simulink model "ASM_AnimationInterface"  (R2024a)
settings: Solver=ode1  StartTime=SIM.tstart.v  StopTime=SIM.tend.v  FixedStep=SIM.StepSize.v  RelTol=1e-3
PostLoadFcn:
  | , if any(exist('dsrtsu_mdlpostloadfcn', 'file') ~= 0), dsrtsu_mdlpostloadfcn('Execute', bdroot); end,
undefined symbols (not defined in the file): a0b2, b98103fe8ad365046cd0, dsmsi, MDL, SIM
libraries: simulink x22, dsmsilib x15, dsmpblib x4, ASM_Environment_lib x1
(part 7 of 7)

== system ASM_AnimationInterface/AnimationInterface/ANIMATION_INTERFACE/Sensors/Line_Sensor_Road_Shape_ContObj_Points ==
  ModelSignals : Inport
  Bus Selector : BusSelector  OutputSignals=Pos_x_Road_Shape_ContObj_Animation_CoorSys_E,Pos_y_Road_Shape_ContObj_Animation_CoorSys_E,Pos_z_Road_Shape_ContObj_Animation_CoorSys_E
  CC : Concatenate  NumInputs=3  Mode=Multidimensional array
  Reshape1 : Reshape  OutputDimensionality=Row vector (2-D)
  Reshape2 : Reshape  OutputDimensionality=Row vector (2-D)
  Reshape3 : Reshape  OutputDimensionality=Row vector (2-D)
  AnimationSignals : Outport  VectorParamsAs1DForOutWhenUnconnected=off
  wires:
  ModelSignals/1 -> Bus Selector/1
  CC/1 -> AnimationSignals/1
  Bus Selector/1 -> Reshape1/1  "<Pos_x_Road_Shape_ContObj_Animation_CoorSys_E>"
  Bus Selector/2 -> Reshape2/1  "<Pos_y_Road_Shape_ContObj_Animation_CoorSys_E>"
  Bus Selector/3 -> Reshape3/1  "<Pos_z_Road_Shape_ContObj_Animation_CoorSys_E>"
  Reshape1/1 -> CC/1
  Reshape2/1 -> CC/2
  Reshape3/1 -> CC/3

== system ASM_AnimationInterface/AnimationInterface/ANIMATION_INTERFACE/Sensors/Line_Sensor_Road_Shape_Line_Points ==
  ModelSignals : Inport
  Bus Selector : BusSelector  OutputSignals=Pos_x_Road_Shape_Line_Animation_CoorSys_E,Pos_y_Road_Shape_Line_Animation_CoorSys_E,Pos_z_Road_Shape_Line_Animation_CoorSys_E
  CC : Concatenate  NumInputs=3  Mode=Multidimensional array
  Reshape1 : Reshape  OutputDimensionality=Row vector (2-D)
  Reshape2 : Reshape  OutputDimensionality=Row vector (2-D)
  Reshape3 : Reshape  OutputDimensionality=Row vector (2-D)
  AnimationSignals : Outport  VectorParamsAs1DForOutWhenUnconnected=off
  wires:
  Bus Selector/3 -> Reshape3/1  "<Pos_z_Road_Shape_Line_Animation_CoorSys_E>"
  Bus Selector/2 -> Reshape2/1  "<Pos_y_Road_Shape_Line_Animation_CoorSys_E>"
  Bus Selector/1 -> Reshape1/1  "<Pos_x_Road_Shape_Line_Animation_CoorSys_E>"
  CC/1 -> AnimationSignals/1
  ModelSignals/1 -> Bus Selector/1
  Reshape1/1 -> CC/1
  Reshape2/1 -> CC/2
  Reshape3/1 -> CC/3

== system ASM_AnimationInterface/AnimationInterface/ANIMATION_INTERFACE/Sensors/Object_Sensor_2D_Points ==
  Transform_In : Inport
  Sw_Sensor_Selector[] : Inport  Port=2
  ObjectSensor2D_1_Animation : Inport  Port=3
  ObjectSensor2D_2_Animation : Inport  Port=4
  ObjectSensor2D_3_Animation : Inport  Port=5
  ObjectSensor2D_4_Animation : Inport  Port=6
  ObjectSensor2D_5_Animation : Inport  Port=7
  ObjectSensor2D_6_Animation : Inport  Port=8
  ObjectSensor2D_7_Animation : Inport  Port=9
  Calc_Object_Sensor_2D_Points : Subsystem
  Multiport Switch : MultiPortSwitch  Inputs=7  SaturateOnIntegerOverflow=off  InputSameDT=off
  Object_Sensor_2D_Transformation1 : Subsystem
  Saturation : Saturate  UpperLimit=7  LowerLimit=1
  AnimationSignals : Outport  VectorParamsAs1DForOutWhenUnconnected=off
  wires:
  Saturation/1 -> Multiport Switch/1
  ObjectSensor2D_7_Animation/1 -> Multiport Switch/8
  ObjectSensor2D_6_Animation/1 -> Multiport Switch/7
  ObjectSensor2D_5_Animation/1 -> Multiport Switch/6
  ObjectSensor2D_4_Animation/1 -> Multiport Switch/5
  Transform_In/1 -> Object_Sensor_2D_Transformation1/1(Transform_In1)
  Object_Sensor_2D_Transformation1/1(Transform_Out) -> Calc_Object_Sensor_2D_Points/1(Transform_In)
  Calc_Object_Sensor_2D_Points/1(AnimationSignals) -> AnimationSignals/1
  ObjectSensor2D_3_Animation/1 -> Multiport Switch/4
  ObjectSensor2D_2_Animation/1 -> Multiport Switch/3
  ObjectSensor2D_1_Animation/1 -> Multiport Switch/2
  Sw_Sensor_Selector[]/1 -> Saturation/1
  Multiport Switch/1 -> Object_Sensor_2D_Transformation1/2(ModelSignals), Calc_Object_Sensor_2D_Points/2(ModelSignals)

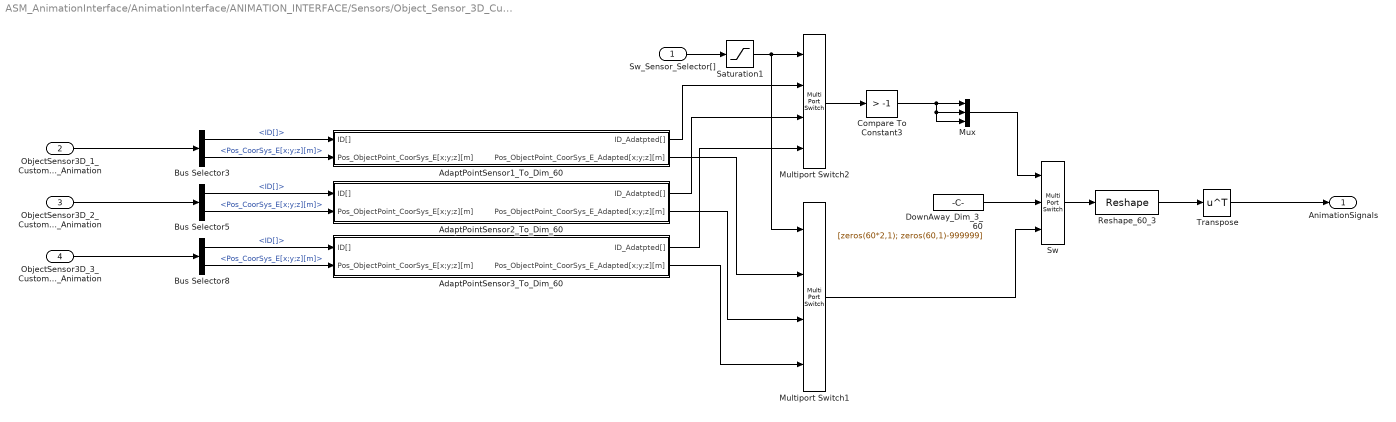
== system ASM_AnimationInterface/AnimationInterface/ANIMATION_INTERFACE/Sensors/Object_Sensor_3D_CustomPoints ==
  Sw_Sensor_Selector[] : Inport
  ObjectSensor3D_1_CustomPoints_Animation : Inport  Port=2
  ObjectSensor3D_2_CustomPoints_Animation : Inport  Port=3
  ObjectSensor3D_3_CustomPoints_Animation : Inport  Port=4
  AdaptPointSensor1_To_Dim_60 : Subsystem
  AdaptPointSensor2_To_Dim_60 : Subsystem
  AdaptPointSensor3_To_Dim_60 : Subsystem
  Bus Selector3 : BusSelector  OutputSignals=ID[],Pos_CoorSys_E[x;y;z][m]
  Bus Selector5 : BusSelector  OutputSignals=ID[],Pos_CoorSys_E[x;y;z][m]
  Bus Selector8 : BusSelector  OutputSignals=ID[],Pos_CoorSys_E[x;y;z][m]
  Compare To Constant3 : simulink/Logic and Bit Operations/Compare To Constant  relop=>  const=-1  OutDataTypeStr=boolean
  DownAway_Dim_3_60 : Constant  Value=[zeros(60*2,1); zeros(60,1)-999999]
  Multiport Switch1 : MultiPortSwitch  SaturateOnIntegerOverflow=off  InputSameDT=off
  Multiport Switch2 : MultiPortSwitch  SaturateOnIntegerOverflow=off  InputSameDT=off
  Mux : Mux  Inputs=3
  Reshape_60_3 : Reshape  OutputDimensionality=Customize  OutputDimensions=[60,3]
  Saturation1 : Saturate  UpperLimit=3  LowerLimit=1
  Sw : MultiPortSwitch  DataPortOrder=Zero-based contiguous  Inputs=2  zeroidx=on  SaturateOnIntegerOverflow=off  InputSameDT=off
  Transpose : Math  Operator=transpose  SignedPower=on
  AnimationSignals : Outport  VectorParamsAs1DForOutWhenUnconnected=off
  wires:
  Transpose/1 -> AnimationSignals/1
  AdaptPointSensor3_To_Dim_60/1(ID_Adatpted[]) -> Multiport Switch2/4
  AdaptPointSensor3_To_Dim_60/2(Pos_ObjectPoint_CoorSys_E_Adapted[x;y;z][m]) -> Multiport Switch1/4
  Multiport Switch1/1 -> Sw/3
  Bus Selector8/2 -> AdaptPointSensor3_To_Dim_60/2(Pos_ObjectPoint_CoorSys_E[x;y;z][m])  "<Pos_CoorSys_E[x;y;z][m]>"
  Bus Selector5/2 -> AdaptPointSensor2_To_Dim_60/2(Pos_ObjectPoint_CoorSys_E[x;y;z][m])  "<Pos_CoorSys_E[x;y;z][m]>"
  Bus Selector5/1 -> AdaptPointSensor2_To_Dim_60/1(ID[])  "<ID[]>"
  Multiport Switch2/1 -> Compare To Constant3/1
  Reshape_60_3/1 -> Transpose/1
  ObjectSensor3D_2_CustomPoints_Animation/1 -> Bus Selector5/1
  ObjectSensor3D_3_CustomPoints_Animation/1 -> Bus Selector8/1
  Bus Selector3/1 -> AdaptPointSensor1_To_Dim_60/1(ID[])  "<ID[]>"
  Bus Selector3/2 -> AdaptPointSensor1_To_Dim_60/2(Pos_ObjectPoint_CoorSys_E[x;y;z][m])  "<Pos_CoorSys_E[x;y;z][m]>"
  ObjectSensor3D_1_CustomPoints_Animation/1 -> Bus Selector3/1
  AdaptPointSensor1_To_Dim_60/1(ID_Adatpted[]) -> Multiport Switch2/2
  AdaptPointSensor1_To_Dim_60/2(Pos_ObjectPoint_CoorSys_E_Adapted[x;y;z][m]) -> Multiport Switch1/2
  Bus Selector8/1 -> AdaptPointSensor3_To_Dim_60/1(ID[])  "<ID[]>"
  Mux/1 -> Sw/1
  Compare To Constant3/1 -> Mux/3, Mux/2, Mux/1
  Sw_Sensor_Selector[]/1 -> Saturation1/1
  DownAway_Dim_3_60/1 -> Sw/2
  Saturation1/1 -> Multiport Switch1/1, Multiport Switch2/1
  Sw/1 -> Reshape_60_3/1
  AdaptPointSensor2_To_Dim_60/2(Pos_ObjectPoint_CoorSys_E_Adapted[x;y;z][m]) -> Multiport Switch1/3
  AdaptPointSensor2_To_Dim_60/1(ID_Adatpted[]) -> Multiport Switch2/3

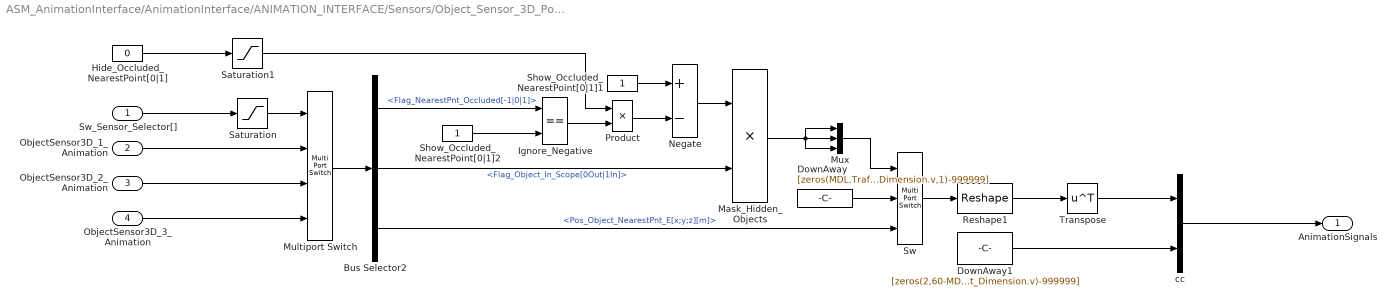
== system ASM_AnimationInterface/AnimationInterface/ANIMATION_INTERFACE/Sensors/Object_Sensor_3D_Points ==
  Sw_Sensor_Selector[] : Inport
  ObjectSensor3D_1_Animation : Inport  Port=2
  ObjectSensor3D_2_Animation : Inport  Port=3
  ObjectSensor3D_3_Animation : Inport  Port=4
  Bus Selector2 : BusSelector  OutputSignals=Flag_NearestPnt_Occluded[-1|0|1],Flag_Object_In_Scope[0Out|1In],Pos_Object_NearestPnt_E[x;y;z][m]
  DownAway : Constant  Value=[zeros(MDL.Traffic.Sensors.ObjectSensor3D_Calculation.Const_Sensor_Output_Dimension.v*2,1); zeros(MDL.Traffic.Sensors.ObjectSensor3D_Calculation.Const_Sensor_Output_Dimension.v,1)-999999]
  DownAway1 : Constant  Value=[zeros(2,60-MDL.Traffic.Sensors.ObjectSensor3D_Calculation.Const_Sensor_Output_Dimension.v); zeros(1,60-MDL.Traffic.Sensors.ObjectSensor3D_Calculation.Const_Sensor_Output_Dimension.v)-999999]
  Hide_Occluded_NearestPoint[0|1] : Constant  Value=0
  Ignore_Negative : RelationalOperator  Operator===  RndMeth=Simplest  InputSameDT=off
  Mask_Hidden_Objects : Product
  Multiport Switch : MultiPortSwitch  SaturateOnIntegerOverflow=off  InputSameDT=off
  Mux : Mux  Inputs=3
  Negate : Sum  Inputs=+-
  Product : Product
  Reshape1 : Reshape  OutputDimensionality=Customize  OutputDimensions=[MDL.Traffic.Sensors.ObjectSensor3D_Calculation.Const_Sensor_Output_Dimension.v,3]
  Saturation : Saturate  UpperLimit=3  LowerLimit=1
  Saturation1 : Saturate  UpperLimit=1  LowerLimit=0
  Show_Occluded_NearestPoint[0|1]1 : Constant
  Show_Occluded_NearestPoint[0|1]2 : Constant
  Sw : MultiPortSwitch  DataPortOrder=Zero-based contiguous  Inputs=2  zeroidx=on  SaturateOnIntegerOverflow=off  InputSameDT=off
  Transpose : Math  Operator=transpose  SignedPower=on
  cc : Concatenate  Mode=Multidimensional array  ConcatenateDimension=2
  AnimationSignals : Outport  VectorParamsAs1DForOutWhenUnconnected=off
  wires:
  ObjectSensor3D_3_Animation/1 -> Multiport Switch/4
  ObjectSensor3D_2_Animation/1 -> Multiport Switch/3
  ObjectSensor3D_1_Animation/1 -> Multiport Switch/2
  Mask_Hidden_Objects/1 -> Mux/2, Mux/1, Mux/3
  Negate/1 -> Mask_Hidden_Objects/1
  Bus Selector2/2 -> Mask_Hidden_Objects/2  "<Flag_Object_In_Scope[0Out|1In]>"
  Ignore_Negative/1 -> Product/2
  Show_Occluded_NearestPoint[0|1]2/1 -> Ignore_Negative/2
  Bus Selector2/1 -> Ignore_Negative/1  "<Flag_NearestPnt_Occluded[-1|0|1]>"
  Show_Occluded_NearestPoint[0|1]1/1 -> Negate/1
  Product/1 -> Negate/2
  Mux/1 -> Sw/1
  Saturation1/1 -> Product/1
  Hide_Occluded_NearestPoint[0|1]/1 -> Saturation1/1
  Saturation/1 -> Multiport Switch/1
  Sw_Sensor_Selector[]/1 -> Saturation/1
  Multiport Switch/1 -> Bus Selector2/1
  Bus Selector2/3 -> Sw/3  "<Pos_Object_NearestPnt_E[x;y;z][m]>"
  DownAway/1 -> Sw/2
  Sw/1 -> Reshape1/1
  Reshape1/1 -> Transpose/1
  Transpose/1 -> cc/1
  DownAway1/1 -> cc/2
  cc/1 -> AnimationSignals/1

== system ASM_AnimationInterface/AnimationInterface/ANIMATION_INTERFACE/Sensors/Object_Sensor_3D_RadarEffect_Points ==
  Sw_Sensor_Selector[] : Inport
  ObjectSensor3D_1_RadarEffects_Animation : Inport  Port=2
  ObjectSensor3D_2_RadarEffects_Animation : Inport  Port=3
  ObjectSensor3D_3_RadarEffects_Animation : Inport  Port=4
  AdaptPointDimensionSensor1 : Subsystem
  AdaptPointDimensionSensor2 : Subsystem
  AdaptPointDimensionSensor3 : Subsystem
  Bus Selector3 : BusSelector  OutputSignals=ID[],Pos_ObjectPoint_CoorSys_E[x;y;z][m]
  Bus Selector5 : BusSelector  OutputSignals=ID[],Pos_ObjectPoint_CoorSys_E[x;y;z][m]
  Bus Selector8 : BusSelector  OutputSignals=ID[],Pos_ObjectPoint_CoorSys_E[x;y;z][m]
  Compare To Constant3 : simulink/Logic and Bit Operations/Compare To Constant  relop=>  const=-1  OutDataTypeStr=boolean
  DownAway : Constant  Value=[zeros(60*2,1); zeros(60,1)-999999]
  Multiport Switch1 : MultiPortSwitch  SaturateOnIntegerOverflow=off  InputSameDT=off
  Multiport Switch2 : MultiPortSwitch  SaturateOnIntegerOverflow=off  InputSameDT=off
  Mux : Mux  Inputs=3
  Reshape1 : Reshape  OutputDimensionality=Customize  OutputDimensions=[60,3]
  Saturation1 : Saturate  UpperLimit=3  LowerLimit=1
  Sw : MultiPortSwitch  DataPortOrder=Zero-based contiguous  Inputs=2  zeroidx=on  SaturateOnIntegerOverflow=off  InputSameDT=off
  Transpose : Math  Operator=transpose  SignedPower=on
  AnimationSignals : Outport  VectorParamsAs1DForOutWhenUnconnected=off
  wires:
  Bus Selector8/2 -> AdaptPointDimensionSensor3/2(Pos_ObjectPoint_CoorSys_E[x;y;z][m])  "<Pos_ObjectPoint_CoorSys_E[x;y;z][m]>"
  Transpose/1 -> AnimationSignals/1
  Reshape1/1 -> Transpose/1
  Mux/1 -> Sw/1
  Sw/1 -> Reshape1/1
  DownAway/1 -> Sw/2
  Compare To Constant3/1 -> Mux/1, Mux/2, Mux/3
  AdaptPointDimensionSensor3/2(Pos_ObjectPoint_CoorSys_E_Adapted[x;y;z][m]) -> Multiport Switch1/4
  AdaptPointDimensionSensor3/1(ID_Adatpted[]) -> Multiport Switch2/4
  Bus Selector5/2 -> AdaptPointDimensionSensor2/2(Pos_ObjectPoint_CoorSys_E[x;y;z][m])  "<Pos_ObjectPoint_CoorSys_E[x;y;z][m]>"
  AdaptPointDimensionSensor2/2(Pos_ObjectPoint_CoorSys_E_Adapted[x;y;z][m]) -> Multiport Switch1/3
  AdaptPointDimensionSensor2/1(ID_Adatpted[]) -> Multiport Switch2/3
  AdaptPointDimensionSensor1/2(Pos_ObjectPoint_CoorSys_E_Adapted[x;y;z][m]) -> Multiport Switch1/2
  AdaptPointDimensionSensor1/1(ID_Adatpted[]) -> Multiport Switch2/2
  Bus Selector3/2 -> AdaptPointDimensionSensor1/2(Pos_ObjectPoint_CoorSys_E[x;y;z][m])  "<Pos_ObjectPoint_CoorSys_E[x;y;z][m]>"
  Bus Selector3/1 -> AdaptPointDimensionSensor1/1(ID[])  "<ID[]>"
  Multiport Switch1/1 -> Sw/3
  Multiport Switch2/1 -> Compare To Constant3/1
  Bus Selector8/1 -> AdaptPointDimensionSensor3/1(ID[])  "<ID[]>"
  Bus Selector5/1 -> AdaptPointDimensionSensor2/1(ID[])  "<ID[]>"
  Sw_Sensor_Selector[]/1 -> Saturation1/1
  Saturation1/1 -> Multiport Switch2/1, Multiport Switch1/1
  ObjectSensor3D_3_RadarEffects_Animation/1 -> Bus Selector8/1
  ObjectSensor3D_2_RadarEffects_Animation/1 -> Bus Selector5/1
  ObjectSensor3D_1_RadarEffects_Animation/1 -> Bus Selector3/1

== system ASM_AnimationInterface/AnimationInterface/ANIMATION_INTERFACE/Sensors/Traffic_Sign_Sensor_Points ==
  ModelSignals : Inport
  Bus Selector2 : BusSelector  OutputSignals=Traffic_Sign_Valid[0|1],Pos_CoorSys_E[x;y;z][m]
  DownAway : Constant  Value=[zeros(2,MDL.Traffic.Sensors.TrafficSignSensorDyn_Calculation.Const_Sensor_Output_Dimension.v); zeros(1,MDL.Traffic.Sensors.TrafficSignSensorDyn_Calculation.Const_Sensor_Output_Dimension.v)-999999]
  DownAway1 : Constant  Value=[zeros(2,60-MDL.Traffic.Sensors.TrafficSignSensorDyn_Calculation.Const_Sensor_Output_Dimension.v); zeros(1,60-MDL.Traffic.Sensors.TrafficSignSensorDyn_Calculation.Const_Sensor_Output_Dimension.v)-999999]
  Reshape1 : Reshape  OutputDimensionality=Customize  OutputDimensions=[3,MDL.Traffic.Sensors.TrafficSignSensorDyn_Calculation.Const_Sensor_Output_Dimension.v]
  Sw : MultiPortSwitch  DataPortOrder=Zero-based contiguous  Inputs=2  zeroidx=on  SaturateOnIntegerOverflow=off  InputSameDT=off
  Trans : Math  Operator=transpose  SignedPower=on
  cc : Concatenate  NumInputs=3  Mode=Multidimensional array  ConcatenateDimension=2
  cc1 : Concatenate  Mode=Multidimensional array  ConcatenateDimension=2
  AnimationSignals : Outport  VectorParamsAs1DForOutWhenUnconnected=off
  wires:
  cc1/1 -> AnimationSignals/1
  Sw/1 -> cc1/1
  DownAway1/1 -> cc1/2
  DownAway/1 -> Sw/2
  Trans/1 -> Sw/1
  cc/1 -> Trans/1
  Reshape1/1 -> Sw/3
  Bus Selector2/1 -> cc/2, cc/1, cc/3  "<Traffic_Sign_Valid[0|1]>"
  Bus Selector2/2 -> Reshape1/1  "<Pos_CoorSys_E[x;y;z][m]>"
  ModelSignals/1 -> Bus Selector2/1

== system ASM_AnimationInterface/AnimationInterface/Fellow_Lights/Coding/SwitchDelay ==
  Turnlight_L : Inport
  Turnlight_R : Inport  Port=2
  Add : Sum
  Compare To Constant : simulink/Logic and Bit Operations/Compare To Constant  relop=>  const=2  OutDataTypeStr=boolean
  Logical Operator1 : Logic  AllPortsSameDT=off  OutDataTypeStr=boolean
  Logical Operator2 : Logic  AllPortsSameDT=off  OutDataTypeStr=boolean
  Logical Operator4 : Logic  AllPortsSameDT=off  OutDataTypeStr=boolean
  Relational Operator3 : RelationalOperator  Operator=>  OutDataTypeStr=boolean  InputSameDT=off
  Switch : Switch  Criteria=u2 > Threshold  SaturateOnIntegerOverflow=off  InputSameDT=off
  Unit Delay{1..3,6} (4 alike) : UnitDelay  SampleTime=-1  HasFrameUpgradeWarning=on
  one : Constant  OutDataTypeStr=uint32
  zero : Constant  Value=0  OutDataTypeStr=uint32
  Turnlight_L_out : Outport  VectorParamsAs1DForOutWhenUnconnected=off
  Turnlight_R_out : Outport  Port=2  VectorParamsAs1DForOutWhenUnconnected=off
  wires:
  Unit Delay6/1 -> Logical Operator4/1
  Unit Delay3/1 -> Logical Operator2/1
  Unit Delay2/1 -> Relational Operator3/2
  Logical Operator1/1 -> Relational Operator3/1, Unit Delay2/1
  Relational Operator3/1 -> Switch/2
  zero/1 -> Switch/1
  Switch/1 -> Unit Delay1/1
  one/1 -> Add/1
  Unit Delay1/1 -> Add/2, Compare To Constant/1
  Add/1 -> Switch/3
  Compare To Constant/1 -> Logical Operator2/2, Logical Operator4/2
  Logical Operator2/1 -> Turnlight_L_out/1
  Logical Operator4/1 -> Turnlight_R_out/1
  Turnlight_L/1 -> Unit Delay3/1, Logical Operator1/1
  Turnlight_R/1 -> Unit Delay6/1, Logical Operator1/2

== system ASM_AnimationInterface/AnimationInterface/Vehicle_Lights/Coding/SwitchDelay ==
  Turnlight_L : Inport
  Turnlight_R : Inport  Port=2
  Add : Sum
  Compare To Constant : simulink/Logic and Bit Operations/Compare To Constant  relop=>  const=2  OutDataTypeStr=boolean
  Logical Operator1 : Logic  AllPortsSameDT=off  OutDataTypeStr=boolean
  Logical Operator2 : Logic  AllPortsSameDT=off  OutDataTypeStr=boolean
  Logical Operator4 : Logic  AllPortsSameDT=off  OutDataTypeStr=boolean
  Relational Operator3 : RelationalOperator  Operator=>  OutDataTypeStr=boolean  InputSameDT=off
  Switch : Switch  Criteria=u2 > Threshold  SaturateOnIntegerOverflow=off  InputSameDT=off
  Unit Delay{1..3,6} (4 alike) : UnitDelay  SampleTime=-1  HasFrameUpgradeWarning=on
  one : Constant  OutDataTypeStr=uint32
  zero : Constant  Value=0  OutDataTypeStr=uint32
  Turnlight_L_out : Outport  VectorParamsAs1DForOutWhenUnconnected=off
  Turnlight_R_out : Outport  Port=2  VectorParamsAs1DForOutWhenUnconnected=off
  wires:
  Unit Delay6/1 -> Logical Operator4/1
  Unit Delay3/1 -> Logical Operator2/1
  Unit Delay2/1 -> Relational Operator3/2
  Logical Operator1/1 -> Relational Operator3/1, Unit Delay2/1
  Relational Operator3/1 -> Switch/2
  zero/1 -> Switch/1
  Switch/1 -> Unit Delay1/1
  one/1 -> Add/1
  Unit Delay1/1 -> Add/2, Compare To Constant/1
  Add/1 -> Switch/3
  Compare To Constant/1 -> Logical Operator2/2, Logical Operator4/2
  Logical Operator2/1 -> Turnlight_L_out/1
  Logical Operator4/1 -> Turnlight_R_out/1
  Turnlight_L/1 -> Unit Delay3/1, Logical Operator1/1
  Turnlight_R/1 -> Unit Delay6/1, Logical Operator1/2

== system ASM_AnimationInterface/AnimationInterface/ANIMATION_INTERFACE/Connection_Settings/Ethernet_TCP/HIL ==
  Tx_Length : Inport
  Tx_Data : Inport  Port=2
  Receive [ETH TCP (Server)\Connection 1] : dsmpblib/Data Inport  Priority=10000
      settings: SourceProductName=dSPACE Model Interface Package for Simulink (MIPS)
  Status [ETH TCP (Server)\Connection 1] : dsmpblib/Data Inport  Priority=10000
      settings: SourceProductName=dSPACE Model Interface Package for Simulink (MIPS)
  Transmit_In [ETH TCP (Server)\Connection 1] : dsmpblib/Data Inport  Priority=10000
      settings: SourceProductName=dSPACE Model Interface Package for Simulink (MIPS)
  Transmit_Out [ETH TCP (Server)\Connection 1] : dsmpblib/Data Outport  Priority=20000
      settings: SourceProductName=dSPACE Model Interface Package for Simulink (MIPS)
  Connected : Outport
  Tx_Sent_bytes : Outport  Port=2
  Rx_Length : Outport  Port=3
  Rx_Data : Outport  Port=4
  wires:
  Receive [ETH TCP (Server)\Connection 1]/2 -> Rx_Data/1
  Receive [ETH TCP (Server)\Connection 1]/1 -> Rx_Length/1
  Transmit_In [ETH TCP (Server)\Connection 1]/1 -> Tx_Sent_bytes/1
  Status [ETH TCP (Server)\Connection 1]/1 -> Connected/1
  Tx_Data/1 -> Transmit_Out [ETH TCP (Server)\Connection 1]/2
  Tx_Length/1 -> Transmit_Out [ETH TCP (Server)\Connection 1]/1

== system ASM_AnimationInterface/AnimationInterface/ANIMATION_INTERFACE/Connection_Settings/Ethernet_TCP/SIL ==
  Tx_Length : Inport
  Tx_Data : Inport  Port=2
  Connected_ : Constant  OutDataTypeStr=Inherit: Inherit via back propagation
  Data Type Conversion : DataTypeConversion  OutDataTypeStr=uint32  SaturateOnIntegerOverflow=off  RndMeth=Floor
  Display : Display
      settings: Format=decimal (Stored Integer)
  dsmsi_eth_tcp_server_BL1 : dsmsilib/Utilities/dsmsi_eth_tcp_server_BL1  paramPort=2017  paramMaximumRxMessageSize=65507  paramBlocking=0  paramEnableReconnectPort=off  paramEnableMaxRxLength=off
      settings: SourceProductName=dSPACE MSI Blockset
  Connected : Outport
  Tx_Sent_bytes : Outport  Port=2
  Rx_Length : Outport  Port=3
  Rx_Data : Outport  Port=4
  wires:
  Tx_Data/1 -> dsmsi_eth_tcp_server_BL1/2
  Tx_Length/1 -> dsmsi_eth_tcp_server_BL1/1
  dsmsi_eth_tcp_server_BL1/1 -> Display/1
  dsmsi_eth_tcp_server_BL1/4 -> Rx_Data/1
  dsmsi_eth_tcp_server_BL1/2 -> Tx_Sent_bytes/1
  Connected_/1 -> Connected/1
  dsmsi_eth_tcp_server_BL1/3 -> Data Type Conversion/1
  Data Type Conversion/1 -> Rx_Length/1

== system ASM_AnimationInterface/AnimationInterface/ANIMATION_INTERFACE/Sensors/Object_Sensor_2D_Points/Calc_Object_Sensor_2D_Points ==
  Transform_In : Inport
  ModelSignals : Inport  Port=2
  Bus Selector2 : BusSelector  OutputSignals=Angle_Hor_Rel[deg],Distance[m],Num_SensorRays_Used[]
  Sensor_Points : Subsystem
  AnimationSignals : Outport  VectorParamsAs1DForOutWhenUnconnected=off
  wires:
  Bus Selector2/1 -> Sensor_Points/2(Angle_Hor_Rel[deg])  "<Angle_Hor_Rel[deg]>"
  Bus Selector2/3 -> Sensor_Points/4(Num_SensorRays_Used[])  "<Num_SensorRays_Used[]>"
  Sensor_Points/1(Translate[x;y;z][m]) -> AnimationSignals/1
  Bus Selector2/2 -> Sensor_Points/3(Distance[m])  "<Distance[m]>"
  Transform_In/1 -> Sensor_Points/1(Transform_In)
  ModelSignals/1 -> Bus Selector2/1

== system ASM_AnimationInterface/AnimationInterface/ANIMATION_INTERFACE/Sensors/Object_Sensor_2D_Points/Object_Sensor_2D_Transformation1 ==
  Transform_In1 : Inport
  ModelSignals : Inport  Port=2
  Bus Selector1 : BusSelector  OutputSignals=Pos_Sensor_Apex_CoorSys_V[x;y;z][m],Angle_z_Orientation_Sensor_CoorSys_V[deg]
  Mux : Mux  Inputs=3
  SensorApex : dsmsilib/dsmsi_simulation_data_objects_BL1  Priority=10001  parameterStr="{\"Version\":1,\"TransformInput\":false,\"EnableInput\":false,\"Objects\":[{\"Name\":\"SensorApex\",\"TypeClass\":{\"Name\":\"Transformation\",\"Class\":1,\"SignalProperty\":null,\"TransformationProperty\":{\"TransformMatrixIn\":true,\"TransformMatrixOut\":true,\"AngleInterpretation\":0,\"TransformationOrder\":0,\"RotationOrder\":0,\"TranslationAsParameter\":false,\"Translation\":\"[0 0 0]\",\"RotationAsParameter\":false,\"Rotation\":\"[0 0 0]\",\"ScalingAsParameter\":true,\"Scaling\":\"[1 1 1]\",\"ObjectsCount\":1},\"PositionAndScaleProperty\":null,\"PositionProperty\":null},\"Children\":[],\"Oid\":1}]}"  evalStr=dsmsi(gcb, 'EvalJson')  sampleTime=-1  globalBlockId=0  objectsBlockId=dsmsi(gcb, 'GetObjectBlockId')  objectsBlockGuiOpen=dsmsi(gcb, 'GetSdoGuiStatus')  dialogIsOpen=0  blockVersion=60  highPrecision=0  validNameBckp=SensorApex
      settings: SourceProductName=dSPACE MSI Blockset
  zero : Constant  Value=0
  Transform_Out : Outport  VectorParamsAs1DForOutWhenUnconnected=off
  wires:
  Bus Selector1/2 -> Mux/1  "<Angle_z_Orientation_Sensor_CoorSys_V[deg]>"
  zero/1 -> Mux/2, Mux/3
  ModelSignals/1 -> Bus Selector1/1
  Transform_In1/1 -> SensorApex/1
  Bus Selector1/1 -> SensorApex/2  "<Pos_Sensor_Apex_CoorSys_V[x;y;z][m]>"
  Mux/1 -> SensorApex/3
  SensorApex/1 -> Transform_Out/1

== system ASM_AnimationInterface/AnimationInterface/ANIMATION_INTERFACE/Sensors/Object_Sensor_3D_CustomPoints/AdaptPointSensor1_To_Dim_60 ==
  ID[] : Inport
  Pos_ObjectPoint_CoorSys_E[x;y;z][m] : Inport  Port=2
  Demux1 : Demux  Outputs=3
  Mux1 : Mux  Inputs=3
  Select_1_60_{1..4} (4 alike) : Selector  InputPortWidth=MDL.Traffic.Sensors.CustomPoints_1.Const_Output_Dimension_Object_Points.v*MDL.Traffic.Sensors.CustomPoints_1.Const_Output_Dimension_Objects.v  IndexOptions=Index vector (dialog)  Indices=[1:60]  OutputSizes=1
  ID_Adatpted[] : Outport  VectorParamsAs1DForOutWhenUnconnected=off
  Pos_ObjectPoint_CoorSys_E_Adapted[x;y;z][m] : Outport  Port=2  VectorParamsAs1DForOutWhenUnconnected=off
  wires:
  Pos_ObjectPoint_CoorSys_E[x;y;z][m]/1 -> Demux1/1
  ID[]/1 -> Select_1_60_1/1
  Select_1_60_1/1 -> ID_Adatpted[]/1
  Select_1_60_2/1 -> Mux1/1
  Demux1/1 -> Select_1_60_2/1
  Demux1/2 -> Select_1_60_3/1
  Select_1_60_3/1 -> Mux1/2
  Select_1_60_4/1 -> Mux1/3
  Demux1/3 -> Select_1_60_4/1
  Mux1/1 -> Pos_ObjectPoint_CoorSys_E_Adapted[x;y;z][m]/1

== system ASM_AnimationInterface/AnimationInterface/ANIMATION_INTERFACE/Sensors/Object_Sensor_3D_CustomPoints/AdaptPointSensor2_To_Dim_60 ==
  ID[] : Inport
  Pos_ObjectPoint_CoorSys_E[x;y;z][m] : Inport  Port=2
  Demux1 : Demux  Outputs=3
  Mux1 : Mux  Inputs=3
  Select_1_60_{1..4} (4 alike) : Selector  InputPortWidth=MDL.Traffic.Sensors.CustomPoints_2.Const_Output_Dimension_Object_Points.v*MDL.Traffic.Sensors.CustomPoints_2.Const_Output_Dimension_Objects.v  IndexOptions=Index vector (dialog)  Indices=[1:60]  OutputSizes=1
  ID_Adatpted[] : Outport  VectorParamsAs1DForOutWhenUnconnected=off
  Pos_ObjectPoint_CoorSys_E_Adapted[x;y;z][m] : Outport  Port=2  VectorParamsAs1DForOutWhenUnconnected=off
  wires:
  Demux1/2 -> Select_1_60_3/1
  Demux1/3 -> Select_1_60_4/1
  ID[]/1 -> Select_1_60_1/1
  Pos_ObjectPoint_CoorSys_E[x;y;z][m]/1 -> Demux1/1
  Mux1/1 -> Pos_ObjectPoint_CoorSys_E_Adapted[x;y;z][m]/1
  Demux1/1 -> Select_1_60_2/1
  Select_1_60_1/1 -> ID_Adatpted[]/1
  Select_1_60_2/1 -> Mux1/1
  Select_1_60_3/1 -> Mux1/2
  Select_1_60_4/1 -> Mux1/3

== system ASM_AnimationInterface/AnimationInterface/ANIMATION_INTERFACE/Sensors/Object_Sensor_3D_CustomPoints/AdaptPointSensor3_To_Dim_60 ==
  ID[] : Inport
  Pos_ObjectPoint_CoorSys_E[x;y;z][m] : Inport  Port=2
  Demux1 : Demux  Outputs=3
  Mux1 : Mux  Inputs=3
  Select_1_60_{1..4} (4 alike) : Selector  InputPortWidth=MDL.Traffic.Sensors.CustomPoints_3.Const_Output_Dimension_Object_Points.v*MDL.Traffic.Sensors.CustomPoints_3.Const_Output_Dimension_Objects.v  IndexOptions=Index vector (dialog)  Indices=[1:60]  OutputSizes=1
  ID_Adatpted[] : Outport  VectorParamsAs1DForOutWhenUnconnected=off
  Pos_ObjectPoint_CoorSys_E_Adapted[x;y;z][m] : Outport  Port=2  VectorParamsAs1DForOutWhenUnconnected=off
  wires:
  Demux1/1 -> Select_1_60_2/1
  Mux1/1 -> Pos_ObjectPoint_CoorSys_E_Adapted[x;y;z][m]/1
  Pos_ObjectPoint_CoorSys_E[x;y;z][m]/1 -> Demux1/1
  ID[]/1 -> Select_1_60_1/1
  Demux1/3 -> Select_1_60_4/1
  Demux1/2 -> Select_1_60_3/1
  Select_1_60_1/1 -> ID_Adatpted[]/1
  Select_1_60_2/1 -> Mux1/1
  Select_1_60_3/1 -> Mux1/2
  Select_1_60_4/1 -> Mux1/3

== system ASM_AnimationInterface/AnimationInterface/ANIMATION_INTERFACE/Sensors/Object_Sensor_3D_RadarEffect_Points/AdaptPointDimensionSensor1 ==
  ID[] : Inport
  Pos_ObjectPoint_CoorSys_E[x;y;z][m] : Inport  Port=2
  Demux1 : Demux  Outputs=3
  Mux1 : Mux  Inputs=3
  Selector{1..4} (4 alike) : Selector  InputPortWidth=MDL.Traffic.Sensors.RadarReflectionPoints_1.Const_Output_Dimension_Objects.v*MDL.Traffic.Sensors.RadarReflectionPoints_1.Const_Output_Dimension_Object_Points.v  IndexOptions=Index vector (dialog)  Indices=[1:60]  OutputSizes=1
  ID_Adatpted[] : Outport  VectorParamsAs1DForOutWhenUnconnected=off
  Pos_ObjectPoint_CoorSys_E_Adapted[x;y;z][m] : Outport  Port=2  VectorParamsAs1DForOutWhenUnconnected=off
  wires:
  Mux1/1 -> Pos_ObjectPoint_CoorSys_E_Adapted[x;y;z][m]/1
  Demux1/3 -> Selector4/1
  Selector4/1 -> Mux1/3
  Selector2/1 -> Mux1/2
  Demux1/2 -> Selector2/1
  Demux1/1 -> Selector1/1
  Selector1/1 -> Mux1/1
  Selector3/1 -> ID_Adatpted[]/1
  ID[]/1 -> Selector3/1
  Pos_ObjectPoint_CoorSys_E[x;y;z][m]/1 -> Demux1/1

== system ASM_AnimationInterface/AnimationInterface/ANIMATION_INTERFACE/Sensors/Object_Sensor_3D_RadarEffect_Points/AdaptPointDimensionSensor2 ==
  ID[] : Inport
  Pos_ObjectPoint_CoorSys_E[x;y;z][m] : Inport  Port=2
  Demux1 : Demux  Outputs=3
  Mux1 : Mux  Inputs=3
  Selector{1..4} (4 alike) : Selector  InputPortWidth=MDL.Traffic.Sensors.RadarReflectionPoints_2.Const_Output_Dimension_Objects.v*MDL.Traffic.Sensors.RadarReflectionPoints_2.Const_Output_Dimension_Object_Points.v  IndexOptions=Index vector (dialog)  Indices=[1:60]  OutputSizes=1
  ID_Adatpted[] : Outport  VectorParamsAs1DForOutWhenUnconnected=off
  Pos_ObjectPoint_CoorSys_E_Adapted[x;y;z][m] : Outport  Port=2  VectorParamsAs1DForOutWhenUnconnected=off
  wires:
  Pos_ObjectPoint_CoorSys_E[x;y;z][m]/1 -> Demux1/1
  ID[]/1 -> Selector3/1
  Selector3/1 -> ID_Adatpted[]/1
  Selector1/1 -> Mux1/1
  Demux1/1 -> Selector1/1
  Demux1/2 -> Selector2/1
  Selector2/1 -> Mux1/2
  Selector4/1 -> Mux1/3
  Demux1/3 -> Selector4/1
  Mux1/1 -> Pos_ObjectPoint_CoorSys_E_Adapted[x;y;z][m]/1

== system ASM_AnimationInterface/AnimationInterface/ANIMATION_INTERFACE/Sensors/Object_Sensor_3D_RadarEffect_Points/AdaptPointDimensionSensor3 ==
  ID[] : Inport
  Pos_ObjectPoint_CoorSys_E[x;y;z][m] : Inport  Port=2
  Demux1 : Demux  Outputs=3
  Mux1 : Mux  Inputs=3
  Selector{1..4} (4 alike) : Selector  InputPortWidth=MDL.Traffic.Sensors.RadarReflectionPoints_3.Const_Output_Dimension_Objects.v*MDL.Traffic.Sensors.RadarReflectionPoints_3.Const_Output_Dimension_Object_Points.v  IndexOptions=Index vector (dialog)  Indices=[1:60]  OutputSizes=1
  ID_Adatpted[] : Outport  VectorParamsAs1DForOutWhenUnconnected=off
  Pos_ObjectPoint_CoorSys_E_Adapted[x;y;z][m] : Outport  Port=2  VectorParamsAs1DForOutWhenUnconnected=off
  wires:
  Mux1/1 -> Pos_ObjectPoint_CoorSys_E_Adapted[x;y;z][m]/1
  Demux1/3 -> Selector4/1
  Selector4/1 -> Mux1/3
  Selector2/1 -> Mux1/2
  Demux1/2 -> Selector2/1
  Demux1/1 -> Selector1/1
  Selector1/1 -> Mux1/1
  Selector3/1 -> ID_Adatpted[]/1
  ID[]/1 -> Selector3/1
  Pos_ObjectPoint_CoorSys_E[x;y;z][m]/1 -> Demux1/1

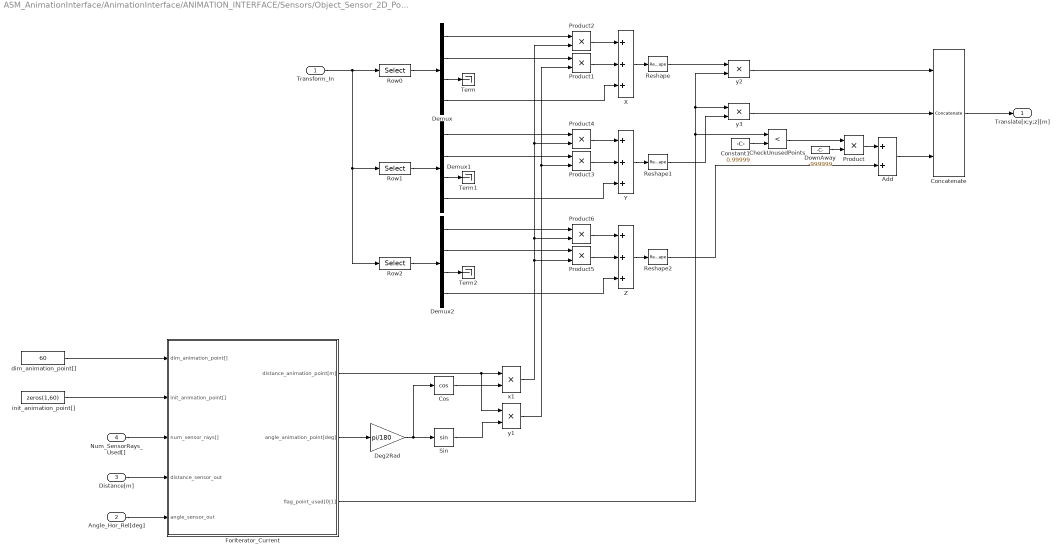
== system ASM_AnimationInterface/AnimationInterface/ANIMATION_INTERFACE/Sensors/Object_Sensor_2D_Points/Calc_Object_Sensor_2D_Points/Sensor_Points ==
  Transform_In : Inport
  Angle_Hor_Rel[deg] : Inport  Port=2
  Distance[m] : Inport  Port=3
  Num_SensorRays_Used[] : Inport  Port=4
  Add : Sum
  CheckUnusedPoints : RelationalOperator  Operator=<  OutDataTypeStr=boolean  InputSameDT=off
  Concatenate : Concatenate  NumInputs=3  Mode=Multidimensional array
  Constant1 : Constant  Value=0.99999
  Cos : Trigonometry  Operator=cos
  Deg2Rad : Gain  Gain=pi/180
  Demux : Demux
  Demux1 : Demux
  Demux2 : Demux
  DownAway : Constant  Value=-999999
  ForIterator_Current : Subsystem  TreatAsAtomicUnit=on
  Product{,1..6} (7 alike) : Product
  Reshape : Reshape  OutputDimensionality=Row vector (2-D)
  Reshape1 : Reshape  OutputDimensionality=Row vector (2-D)
  Reshape2 : Reshape  OutputDimensionality=Row vector (2-D)
  Row0 : Selector  NumberOfDimensions=2  IndexMode=Zero-based  InputPortWidth=3  IndexOptions=Index vector (dialog),Index vector (dialog)  Indices=0,-1  OutputSizes=1,1
  Row1 : Selector  NumberOfDimensions=2  IndexMode=Zero-based  InputPortWidth=3  IndexOptions=Index vector (dialog),Index vector (dialog)  Indices=1,-1  OutputSizes=1,1
  Row2 : Selector  NumberOfDimensions=2  IndexMode=Zero-based  InputPortWidth=3  IndexOptions=Index vector (dialog),Index vector (dialog)  Indices=2,-1  OutputSizes=1,1
  Sin : Trigonometry
  Term : Terminator
  Term1 : Terminator
  Term2 : Terminator
  X : Sum  Inputs=+++
  Y : Sum  Inputs=+++
  Z : Sum  Inputs=+++
  dim_animation_point[] : Constant  Value=60
  init_animation_point[] : Constant  Value=zeros(1,60)  VectorParams1D=off
  x1 : Product
  y1 : Product
  y2 : Product
  y3 : Product
  Translate[x;y;z][m] : Outport  VectorParamsAs1DForOutWhenUnconnected=off
  wires:
  CheckUnusedPoints/1 -> Product/1
  Constant1/1 -> CheckUnusedPoints/2
  Product/1 -> Add/1
  DownAway/1 -> Product/2
  Add/1 -> Concatenate/3
  Reshape2/1 -> Add/2
  ForIterator_Current/3(flag_point_used[0|1]) -> CheckUnusedPoints/1, y3/1, y2/2
  Z/1 -> Reshape2/1
  Demux2/4 -> Z/3
  Product5/1 -> Z/2
  Product6/1 -> Z/1
  Demux2/3 -> Term2/1
  Demux2/2 -> Product5/1
  Demux2/1 -> Product6/1
  Row2/1 -> Demux2/1
  Y/1 -> Reshape1/1
  X/1 -> Reshape/1
  Concatenate/1 -> Translate[x;y;z][m]/1
  Demux1/4 -> Y/3
  Product3/1 -> Y/2
  Product4/1 -> Y/1
  Demux1/3 -> Term1/1
  Demux1/2 -> Product3/1
  Demux1/1 -> Product4/1
  Row1/1 -> Demux1/1
  Demux/4 -> X/3
  Product1/1 -> X/2
  Product2/1 -> X/1
  Demux/3 -> Term/1
  Demux/2 -> Product1/1
  Demux/1 -> Product2/1
  Row0/1 -> Demux/1
  y1/1 -> Product1/2, Product3/2
  x1/1 -> Product2/2, Product4/2, Product6/2, Product5/2
  Transform_In/1 -> Row0/1, Row1/1, Row2/1
  Sin/1 -> y1/2
  Cos/1 -> x1/2
  ForIterator_Current/1(distance_animation_point[m]) -> x1/1, y1/1
  Deg2Rad/1 -> Sin/1, Cos/1
  ForIterator_Current/2(angle_animation_point[deg]) -> Deg2Rad/1
  Num_SensorRays_Used[]/1 -> ForIterator_Current/3(num_sensor_rays[])
  dim_animation_point[]/1 -> ForIterator_Current/1(dim_animation_point[])
  Distance[m]/1 -> ForIterator_Current/4(distance_sensor_out)
  Angle_Hor_Rel[deg]/1 -> ForIterator_Current/5(angle_sensor_out)
  Reshape/1 -> y2/1
  Reshape1/1 -> y3/2
  init_animation_point[]/1 -> ForIterator_Current/2(init_animation_point[])
  y2/1 -> Concatenate/1
  y3/1 -> Concatenate/2

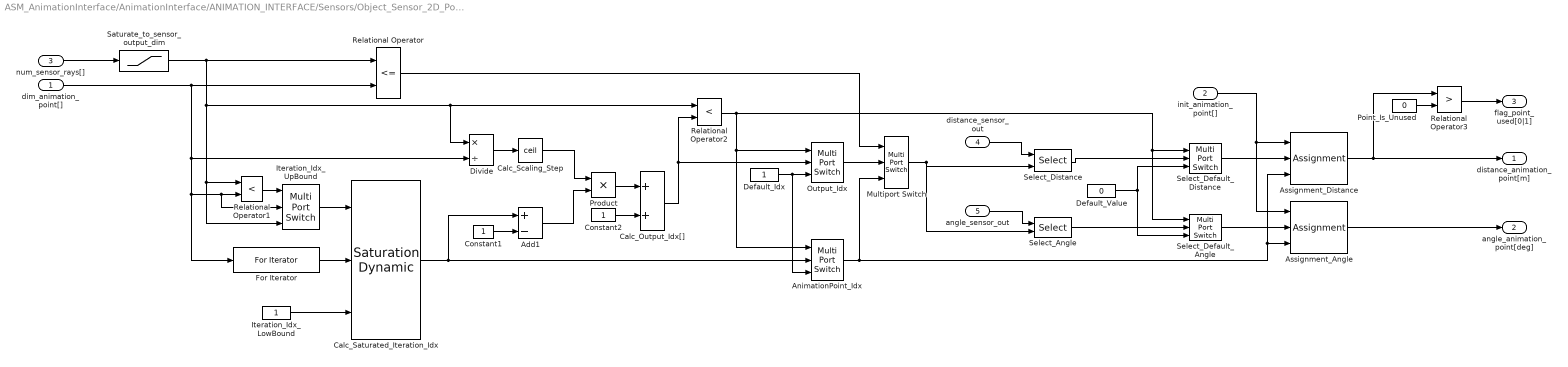
== system ASM_AnimationInterface/AnimationInterface/ANIMATION_INTERFACE/Sensors/Object_Sensor_2D_Points/Calc_Object_Sensor_2D_Points/Sensor_Points/ForIterator_Current ==
  dim_animation_point[] : Inport
  init_animation_point[] : Inport  Port=2
  num_sensor_rays[] : Inport  Port=3
  distance_sensor_out : Inport  Port=4
  angle_sensor_out : Inport  Port=5
  Add1 : Sum  Inputs=+-
  AnimationPoint_Idx : MultiPortSwitch  DataPortOrder=Zero-based contiguous  Inputs=2  zeroidx=on  SaturateOnIntegerOverflow=off  InputSameDT=off
  Assignment_Angle : Assignment  IndexOptions=Index vector (port)  Indices=1  OutputSizes=1
  Assignment_Distance : Assignment  IndexOptions=Index vector (port)  Indices=1  OutputSizes=1
  Calc_Output_Idx[] : Sum
  Calc_Saturated_Iteration_Idx : simulink/Discontinuities/Saturation Dynamic  OutMin=[]  OutMax=[]  OutDataTypeStr=Inherit: Same as second input  OutDataType=fixdt(1, 16)  OutScaling=2^-10  DoSatur=off
  Calc_Scaling_Step : Rounding  Operator=ceil
  Constant1 : Constant
  Constant2 : Constant
  Default_Idx : Constant
  Default_Value : Constant  Value=0
  Divide : Product  Inputs=*/
  For Iterator : ForIterator  ResetStates=reset  IterationSource=external  IterationLimit=36
  Iteration_Idx_LowBound : Constant
  Iteration_Idx_UpBound : MultiPortSwitch  DataPortOrder=Zero-based contiguous  Inputs=2  zeroidx=on  SaturateOnIntegerOverflow=off  InputSameDT=off
  Multiport Switch : MultiPortSwitch  DataPortOrder=Zero-based contiguous  Inputs=2  zeroidx=on  SaturateOnIntegerOverflow=off  InputSameDT=off
  Output_Idx : MultiPortSwitch  DataPortOrder=Zero-based contiguous  Inputs=2  zeroidx=on  SaturateOnIntegerOverflow=off  InputSameDT=off
  Point_Is_Unused : Constant  Value=0
  Product : Product
  Relational Operator : RelationalOperator  Operator=<=  OutDataTypeStr=boolean  InputSameDT=off
  Relational Operator1 : RelationalOperator  Operator=<  OutDataTypeStr=boolean  InputSameDT=off
  Relational Operator2 : RelationalOperator  Operator=<  OutDataTypeStr=boolean  InputSameDT=off
  Relational Operator3 : RelationalOperator  Operator=>  OutDataTypeStr=boolean  InputSameDT=off
  Saturate_to_sensor_output_dim : Saturate  UpperLimit=MDL.Traffic.Sensors.ObjectSensor2D_Calculation.Const_Sensor_Output_Dimension.v  LowerLimit=1
  Select_Angle : Selector  InputPortWidth=MDL.Traffic.Sensors.ObjectSensor2D_Calculation.Const_Sensor_Output_Dimension.v  IndexOptions=Starting index (port)  Indices=[1 3]  OutputSizes=1
  Select_Default_Angle : MultiPortSwitch  DataPortOrder=Zero-based contiguous  Inputs=2  zeroidx=on  SaturateOnIntegerOverflow=off  InputSameDT=off
  Select_Default_Distance : MultiPortSwitch  DataPortOrder=Zero-based contiguous  Inputs=2  zeroidx=on  SaturateOnIntegerOverflow=off  InputSameDT=off
  Select_Distance : Selector  InputPortWidth=MDL.Traffic.Sensors.ObjectSensor2D_Calculation.Const_Sensor_Output_Dimension.v  IndexOptions=Starting index (port)  Indices=[1 3]  OutputSizes=1
  distance_animation_point[m] : Outport  InitialOutput=0  VectorParamsAs1DForOutWhenUnconnected=off
  angle_animation_point[deg] : Outport  Port=2  InitialOutput=0  VectorParamsAs1DForOutWhenUnconnected=off
  flag_point_used[0|1] : Outport  Port=3  InitialOutput=0  VectorParamsAs1DForOutWhenUnconnected=off
  wires:
  Relational Operator3/1 -> flag_point_used[0|1]/1
  Select_Default_Angle/1 -> Assignment_Angle/2
  Default_Value/1 -> Select_Default_Angle/3, Select_Default_Distance/3
  Select_Default_Distance/1 -> Assignment_Distance/2
  num_sensor_rays[]/1 -> Saturate_to_sensor_output_dim/1
  dim_animation_point[]/1 -> Relational Operator/2, Divide/2, Relational Operator1/2, Iteration_Idx_UpBound/2, For Iterator/1
  Divide/1 -> Calc_Scaling_Step/1
  Calc_Saturated_Iteration_Idx/1 -> AnimationPoint_Idx/2, Add1/1
  Calc_Scaling_Step/1 -> Product/1
  Constant1/1 -> Add1/2
  Product/1 -> Calc_Output_Idx[]/1
  Constant2/1 -> Calc_Output_Idx[]/2
  Add1/1 -> Product/2
  Calc_Output_Idx[]/1 -> Relational Operator2/2, Output_Idx/2
  Default_Idx/1 -> Output_Idx/3, AnimationPoint_Idx/3
  Relational Operator2/1 -> Select_Default_Angle/1, Select_Default_Distance/1, Output_Idx/1, AnimationPoint_Idx/1
  Relational Operator1/1 -> Iteration_Idx_UpBound/1
  Iteration_Idx_UpBound/1 -> Calc_Saturated_Iteration_Idx/1
  Iteration_Idx_LowBound/1 -> Calc_Saturated_Iteration_Idx/3
  For Iterator/1 -> Calc_Saturated_Iteration_Idx/2
  AnimationPoint_Idx/1 -> Assignment_Distance/3, Assignment_Angle/3, Multiport Switch/3
  Multiport Switch/1 -> Select_Distance/2, Select_Angle/2
  Output_Idx/1 -> Multiport Switch/2
  Relational Operator/1 -> Multiport Switch/1
  Select_Angle/1 -> Select_Default_Angle/2
  Select_Distance/1 -> Select_Default_Distance/2
  distance_sensor_out/1 -> Select_Distance/1
  angle_sensor_out/1 -> Select_Angle/1
  Assignment_Angle/1 -> angle_animation_point[deg]/1
  Assignment_Distance/1 -> Relational Operator3/1, distance_animation_point[m]/1
  init_animation_point[]/1 -> Assignment_Angle/1, Assignment_Distance/1
  Saturate_to_sensor_output_dim/1 -> Relational Operator2/1, Divide/1, Relational Operator1/1, Iteration_Idx_UpBound/3, Relational Operator/1
  Point_Is_Unused/1 -> Relational Operator3/2

== matlab function ASM_AnimationInterface/AnimationInterface/ANIMATION_INTERFACE/Bounding_Boxes/EnableBoxVisualization/Move_Unused_Bounding_Boxes ==
  data: pos_x_out output; pos_y_out output; pos_z_out output; angle_x_out output; angle_y_out output; angle_z_out output; length_out output; width_out output; height_out output; pos_x_in input; pos_y_in input; pos_z_in input; angle_x_in input; angle_y_in input; angle_z_in input; length_in input; width_in input; height_in input
function [pos_x_out, pos_y_out, pos_z_out, angle_x_out, angle_y_out, angle_z_out, length_out, width_out, height_out] = ...
    Move_Unused_Bounding_Boxes(pos_x_in, pos_y_in, pos_z_in, angle_x_in, angle_y_in, angle_z_in, length_in, width_in, height_in)

pos_x_out   = pos_x_in;
pos_y_out   = pos_y_in;
pos_z_out   = pos_z_in;

angle_x_out = angle_x_in;
angle_y_out = angle_y_in;
angle_z_out = angle_z_in;

length_out  = length_in;
width_out   = width_in;
height_out  = height_in;

num_objects = length(pos_x_in);

for i = 1:num_objects
    if length_in(i) == 0.0
        % Move bounding box to [x, y, z] = [-1e9, -1e9, -1e9] since object
        % is not available
        pos_x_out(i) = -1e9;
        pos_y_out(i) = -1e9;
        pos_z_out(i) = -1e9;

        % Scale down bounding box
        length_out(i) = 0.1;
        width_out(i)  = 0.1;
        height_out(i) = 0.1;
    end
end
